simulink model "open_loop"  (R2024b)
settings: Solver=VariableStepAuto  StartTime=0.0  StopTime=0.05  RelTol=1e-3
libraries: spsCurrentMeasurementLib x6, spsVoltageMeasurementLib x6, spsSeriesRLCBranchLib x3, spsDCVoltageSourceLib x1, spsDiodeLib x1, spsMosfetLib x1, sps_lib x1
settings Model: Creator=manas  LastModifiedBy=manas

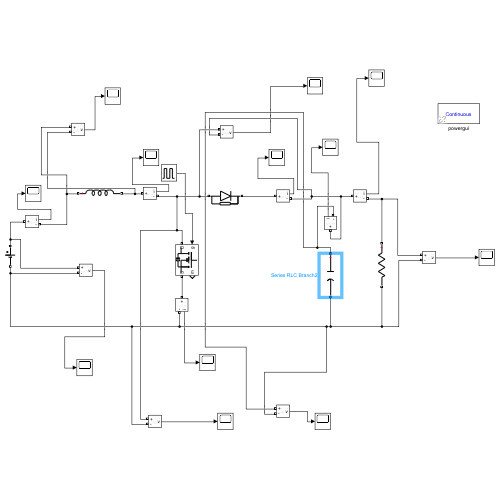
[thumbnail: Simulink's stored preview of the top-level diagram]
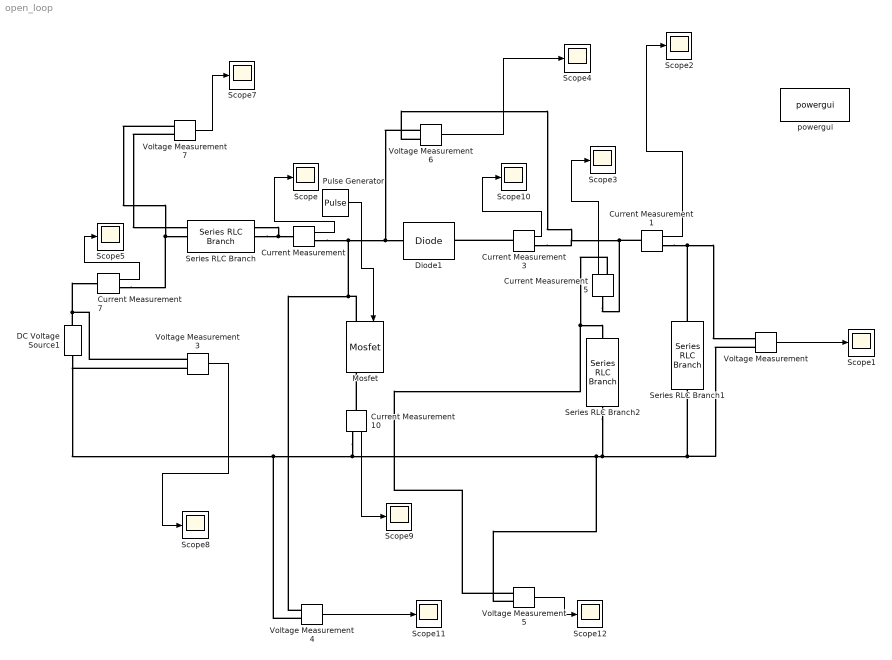
== system open_loop ==
  Current Measurement{,1,3,5,7,10} (6 alike) : spsCurrentMeasurementLib/Current Measurement  PhasorSimulation=off  OutputType=Complex  PSBequivalent=0
  DC Voltage Source1 : spsDCVoltageSourceLib/DC Voltage Source  Amplitude=12  Measurements=None
  Diode1 : spsDiodeLib/Diode  Ron=0.001  Lon=0  Vf=0.8  IC=0  UseSnubber=0  Rs=500  Cs=250e-9  Measurements=off
  Mosfet : spsMosfetLib/Mosfet  Ron=0.1  Lon=0  Rd=0.01  Vfd=0  IC=0  Rs=1e5  Cs=inf  Measurements=on
  Pulse Generator : DiscretePulseGenerator  PulseType=Time based  Period=40e-6  PulseWidth=40
  Scope{,1..5,7..12} (12 alike) : Scope
  Series RLC Branch : spsSeriesRLCBranchLib/Series RLC Branch  LConnTagsString=__new0  RConnTagsString=__new0  BranchType=L  Resistance=1  Inductance=76.8e-6  SetiL0=off  InitialCurrent=0  Capacitance=1e-6  Setx0=off  InitialVoltage=0  Measurements=None
  Series RLC Branch1 : spsSeriesRLCBranchLib/Series RLC Branch  LConnTagsString=__new0  RConnTagsString=__new0  BranchType=R  Resistance=4  Inductance=1e-3  SetiL0=off  InitialCurrent=0  Capacitance=1e-6  Setx0=off  InitialVoltage=0  Measurements=None
  Series RLC Branch2 : spsSeriesRLCBranchLib/Series RLC Branch  LConnTagsString=__new0  RConnTagsString=__new0  BranchType=C  Resistance=1  Inductance=1e-3  SetiL0=off  InitialCurrent=0  Capacitance=400e-6  Setx0=off  InitialVoltage=0  Measurements=None
  Voltage Measurement{,3..7} (6 alike) : spsVoltageMeasurementLib/Voltage Measurement  PhasorSimulation=off  OutputType=Complex  PSBequivalent=0
  powergui : sps_lib/powergui  Priority=1  SimulationMode=Continuous  SampleTime=50e-6  frequency=60  Iterations=50  frequencyindice=0  Pbase=100e6  ErrMax=1e-4  UnitsV=kV  UnitsW=MW  buscounter=0  FunctionMessages=off  echomessages=off  EnableUseOfTLC=off  CurrentSourceSwitches=off  DisableSnubberDevices=off  DisableRonSwitches=off  DisableVfSwitches=off  DisplayEquations=off  AutomaticDiscreteSolvers=off  SolverType=Tustin/Backward Euler (TBE)  Interpol=off  ExternalGateDelay=off  methode=off  Ts=100  x0status=blocks  SPID=on  SwTol=0  HookPort=off  NonlinearTolerance=1e-4  nMaxIteration=100  ContinueOnMaxIteration=off  RestoreLinks=warning  ResistiveCurrentMeasurement=off  Frange=[0:2:500]  Ylog=off  Xlog=on  ShowGrid=off  save=off  variable=ZData  structure=0  ZoomFFT=off  StartTime=0.0  cycles=1  DisplayStyle=1  fundamental=60  FreqAxis=off  MaxFrequency=1000  frequencyindicesteady=1  RmsSteady=1  display=off
  wires:
  Voltage Measurement/1 -> Scope1/1
  Pulse Generator/1 -> Mosfet/1
  Current Measurement/1 -> Scope/1
  Current Measurement1/1 -> Scope2/1
  Voltage Measurement7/1 -> Scope7/1
  Voltage Measurement6/1 -> Scope4/1
  Voltage Measurement5/1 -> Scope12/1
  Voltage Measurement4/1 -> Scope11/1
  Current Measurement10/1 -> Scope9/1
  Current Measurement5/1 -> Scope3/1
  Current Measurement3/1 -> Scope10/1
  Current Measurement7/1 -> Scope5/1
  Voltage Measurement3/1 -> Scope8/1
  connections:
  Voltage Measurement7/LConn1 -- Current Measurement7/RConn1 -- Series RLC Branch/LConn1
  Mosfet/LConn1 -- Current Measurement/RConn1 -- Voltage Measurement6/LConn1 -- Diode1/LConn1 -- Voltage Measurement4/LConn1
  Series RLC Branch1/LConn1 -- Voltage Measurement/LConn1 -- Current Measurement1/RConn1
  Series RLC Branch2/RConn1 -- Current Measurement10/RConn1 -- Voltage Measurement3/LConn2 -- DC Voltage Source1/LConn1 -- Voltage Measurement4/LConn2 -- Voltage Measurement5/LConn2 -- Voltage Measurement/LConn2 -- Series RLC Branch1/RConn1
  Series RLC Branch/RConn1 -- Voltage Measurement7/LConn2 -- Current Measurement/LConn1
  Current Measurement5/LConn1 -- Voltage Measurement6/LConn2 -- Current Measurement3/RConn1 -- Current Measurement1/LConn1
  Current Measurement10/LConn1 -- Mosfet/RConn1
  Voltage Measurement5/LConn1 -- Current Measurement5/RConn1 -- Series RLC Branch2/LConn1
  Current Measurement3/LConn1 -- Diode1/RConn1
  DC Voltage Source1/RConn1 -- Current Measurement7/LConn1 -- Voltage Measurement3/LConn1
